simulink model "fft_biplex_real_4x_delay_bram_test"  (Simulink 7.4)
settings: Solver=VariableStepDiscrete  StartTime=0.0  StopTime=256  RelTol=1e-3
libraries: xbsIndex_r4 x596, casper_library_misc x36, casper_library_delays x8, casper_library_ffts_twiddle x1, simulink x1
(part 4 of 6)

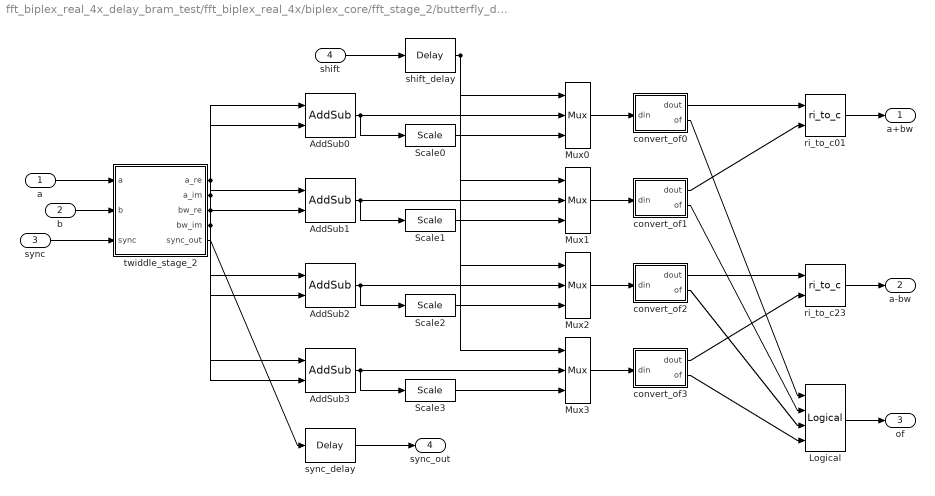
== system fft_biplex_real_4x_delay_bram_test/fft_biplex_real_4x/biplex_core/fft_stage_2/butterfly_direct ==
  a : Inport  OutDataType=sfix(16)  OutScaling=2^0
  b : Inport  Port=2  OutDataType=sfix(16)  OutScaling=2^0
  sync : Inport  Port=3  OutDataType=sfix(16)  OutScaling=2^0
  shift : Inport  Port=4  OutDataType=sfix(16)  OutScaling=2^0
  AddSub0 : xbsIndex_r4/AddSub  mode=Addition  use_carryin=off  use_carryout=off  en=off  latency=1  precision=Full  arith_type=Unsigned  n_bits=16  bin_pt=14  quantization=Truncate  overflow=Wrap  dbl_ovrd=off  use_behavioral_HDL=on  hw_selection=Fabric  pipelined=off  block_type=addsub
  AddSub1 : xbsIndex_r4/AddSub  mode=Addition  use_carryin=off  use_carryout=off  en=off  latency=1  precision=Full  arith_type=Unsigned  n_bits=16  bin_pt=14  quantization=Truncate  overflow=Wrap  dbl_ovrd=off  use_behavioral_HDL=on  hw_selection=Fabric  pipelined=off  block_type=addsub
  AddSub2 : xbsIndex_r4/AddSub  mode=Subtraction  use_carryin=off  use_carryout=off  en=off  latency=1  precision=Full  arith_type=Unsigned  n_bits=16  bin_pt=14  quantization=Truncate  overflow=Wrap  dbl_ovrd=off  use_behavioral_HDL=on  hw_selection=Fabric  pipelined=off  block_type=addsub
  AddSub3 : xbsIndex_r4/AddSub  mode=Subtraction  use_carryin=off  use_carryout=off  en=off  latency=1  precision=Full  arith_type=Unsigned  n_bits=16  bin_pt=14  quantization=Truncate  overflow=Wrap  dbl_ovrd=off  use_behavioral_HDL=on  hw_selection=Fabric  pipelined=off  block_type=addsub
  Logical : xbsIndex_r4/Logical  logical_function=OR  inputs=4  en=off  latency=0  precision=Full  arith_type=Unsigned  n_bits=16  bin_pt=0  align_bp=on  dbl_ovrd=off  block_type=logical
      settings: block_version=11.4
  Mux{0..3} (4 alike) : xbsIndex_r4/Mux  inputs=2  en=off  latency=1  precision=Full  arith_type=Unsigned  n_bits=16  bin_pt=14  quantization=Truncate  overflow=Wrap  dbl_ovrd=off  block_type=mux
      settings: block_version=11.4
  Scale{0..3} (4 alike) : xbsIndex_r4/Scale  scale_factor=-1  dbl_ovrd=off  block_type=scale
  convert_of0 : Subsystem  AncestorBlock=casper_library_misc/convert_of  mask(convert_of){bit_width_i=18, binary_point_i=16, bit_width_o=16, binary_point_o=15, latency=2, overflow=Saturate, quantization=Truncate}
      mask prompts: bit_width_i "Bit Width In"; binary_point_i "Binary Point In"; bit_width_o "Bit Width Out"; binary_point_o "Binary Point Out"; overflow "Overflow Behaviour"; quantization "Quantization Behaviour"
      mask help:
      | Converts from one 2's complement bit-width
      | and/or binary point position to another.
      | Includes underflow/overflow indicator.
      mask init: same as fft_biplex_real_4x_delay_bram_test/fft_biplex_real_4x/biplex_core/fft_stage_1/butterfly_direct/convert_of0
      settings: AttributesFormatString=[18,16]->[16,15]
      mask StyleString: edit,edit,edit,edit,edit,popup(Wrap|Saturate|Error),popup(Truncate|Round  (unbiased: +/- Inf)|Round  (unbiased: even values))
  convert_of1 : Subsystem  AncestorBlock=casper_library_misc/convert_of  mask(convert_of){bit_width_i=18, binary_point_i=16, bit_width_o=16, binary_point_o=15, latency=2, overflow=Saturate, quantization=Truncate}
      mask prompts: bit_width_i "Bit Width In"; binary_point_i "Binary Point In"; bit_width_o "Bit Width Out"; binary_point_o "Binary Point Out"; overflow "Overflow Behaviour"; quantization "Quantization Behaviour"
      mask help:
      | Converts from one 2's complement bit-width
      | and/or binary point position to another.
      | Includes underflow/overflow indicator.
      mask init: same as fft_biplex_real_4x_delay_bram_test/fft_biplex_real_4x/biplex_core/fft_stage_1/butterfly_direct/convert_of0
      settings: AttributesFormatString=[18,16]->[16,15]
      mask StyleString: edit,edit,edit,edit,edit,popup(Wrap|Saturate|Error),popup(Truncate|Round  (unbiased: +/- Inf)|Round  (unbiased: even values))
  convert_of2 : Subsystem  AncestorBlock=casper_library_misc/convert_of  mask(convert_of){bit_width_i=18, binary_point_i=16, bit_width_o=16, binary_point_o=15, latency=2, overflow=Saturate, quantization=Truncate}
      mask prompts: bit_width_i "Bit Width In"; binary_point_i "Binary Point In"; bit_width_o "Bit Width Out"; binary_point_o "Binary Point Out"; overflow "Overflow Behaviour"; quantization "Quantization Behaviour"
      mask help:
      | Converts from one 2's complement bit-width
      | and/or binary point position to another.
      | Includes underflow/overflow indicator.
      mask init: same as fft_biplex_real_4x_delay_bram_test/fft_biplex_real_4x/biplex_core/fft_stage_1/butterfly_direct/convert_of0
      settings: AttributesFormatString=[18,16]->[16,15]
      mask StyleString: edit,edit,edit,edit,edit,popup(Wrap|Saturate|Error),popup(Truncate|Round  (unbiased: +/- Inf)|Round  (unbiased: even values))
  convert_of3 : Subsystem  AncestorBlock=casper_library_misc/convert_of  mask(convert_of){bit_width_i=18, binary_point_i=16, bit_width_o=16, binary_point_o=15, latency=2, overflow=Saturate, quantization=Truncate}
      mask prompts: bit_width_i "Bit Width In"; binary_point_i "Binary Point In"; bit_width_o "Bit Width Out"; binary_point_o "Binary Point Out"; overflow "Overflow Behaviour"; quantization "Quantization Behaviour"
      mask help:
      | Converts from one 2's complement bit-width
      | and/or binary point position to another.
      | Includes underflow/overflow indicator.
      mask init: same as fft_biplex_real_4x_delay_bram_test/fft_biplex_real_4x/biplex_core/fft_stage_1/butterfly_direct/convert_of0
      settings: AttributesFormatString=[18,16]->[16,15]
      mask StyleString: edit,edit,edit,edit,edit,popup(Wrap|Saturate|Error),popup(Truncate|Round  (unbiased: +/- Inf)|Round  (unbiased: even values))
  ri_to_c01 : casper_library_misc/ri_to_c  SystemSampleTime=-1
  ri_to_c23 : casper_library_misc/ri_to_c  SystemSampleTime=-1
  shift_delay : xbsIndex_r4/Delay  en=off  latency=1  dbl_ovrd=off  reg_retiming=off  block_type=delay
      settings: block_version=11.4
  sync_delay : xbsIndex_r4/Delay  en=off  latency=4  dbl_ovrd=off  reg_retiming=on  block_type=delay
      settings: block_version=11.4
  twiddle_stage_2 : Subsystem  AncestorBlock=casper_library_ffts_twiddle/twiddle_stage_2  mask(twiddle_pass_through){FFTSize=5, input_bit_width=16, add_latency=1, mult_latency=3, bram_latency=1, conv_latency=2, opt_target=multipliers}
      mask prompts: FFTSize "FFT Size (2^?)"; input_bit_width "Input Bit Width"; add_latency "Add Latency"; mult_latency "Mult Latency"; bram_latency "BRAM Latency"; conv_latency "Convert latency"; opt_target "Use less"
      mask help:
      | Used in FFT library. Used when coefficients
      | are 2^0 i.e just pass data through without delays
      mask init:
      | set_param(gcb,'LinkStatus','inactive');
      | if(strcmp(opt_target, 'logic')), 
      |     lat = add_latency;
      |     lat_str = 'add_latency';
      | else,
      |     lat = add_latency*2;
      |     lat_str = 'add_latency*2';
      | end
      | set_param([gcb,'/delay0'], 'latency', ...
      |     ['bram_latency+mult_latency+conv_latency+',lat_str]);
      | set_param([gcb,'/delay1'], 'latency', ...
      |     ['bram_latency+mult_latency+conv_latency+',lat_str]);
      | set_param([gcb,'/mux0'], 'latency', ...
      |     num2str(mult_latency+conv_latency+lat));
      | set_param([gcb,'/mux1'], 'latency', ...
      |     num2str(mult_latency+conv_latency+lat));
      | set_param([gcb,'/delay6'], 'latency', ...
      |     ['mult_latency+conv_latency+',lat_str]);
      mask StyleString: edit,edit,edit,edit,edit,edit,popup(logic|multipliers)
  a+bw : Outport  OutDataType=sfix(16)  OutScaling=2^0
  a-bw : Outport  Port=2  OutDataType=sfix(16)  OutScaling=2^0
  of : Outport  Port=3  OutDataType=sfix(16)  OutScaling=2^0
  sync_out : Outport  Port=4
  wires:
  a/1 -> twiddle_stage_2/1(a)
  b/1 -> twiddle_stage_2/2(b)
  sync/1 -> twiddle_stage_2/3(sync)
  twiddle_stage_2/1(a_re) -> AddSub0/1, AddSub2/1
  twiddle_stage_2/2(a_im) -> AddSub1/1, AddSub3/1
  twiddle_stage_2/3(bw_re) -> AddSub0/2, AddSub2/2
  twiddle_stage_2/4(bw_im) -> AddSub1/2, AddSub3/2
  twiddle_stage_2/5(sync_out) -> sync_delay/1
  shift/1 -> shift_delay/1
  shift_delay/1 -> Mux0/1, Mux1/1, Mux2/1, Mux3/1
  AddSub0/1 -> Mux0/2, Scale0/1
  AddSub1/1 -> Mux1/2, Scale1/1
  AddSub2/1 -> Mux2/2, Scale2/1
  AddSub3/1 -> Mux3/2, Scale3/1
  Scale0/1 -> Mux0/3
  Scale1/1 -> Mux1/3
  Scale2/1 -> Mux2/3
  Scale3/1 -> Mux3/3
  Mux0/1 -> convert_of0/1(din)
  Mux1/1 -> convert_of1/1(din)
  Mux2/1 -> convert_of2/1(din)
  Mux3/1 -> convert_of3/1(din)
  convert_of0/1(dout) -> ri_to_c01/1
  convert_of1/1(dout) -> ri_to_c01/2
  convert_of2/1(dout) -> ri_to_c23/1
  convert_of3/1(dout) -> ri_to_c23/2
  convert_of0/2(of) -> Logical/1
  convert_of1/2(of) -> Logical/2
  convert_of2/2(of) -> Logical/3
  convert_of3/2(of) -> Logical/4
  ri_to_c01/1 -> a+bw/1
  ri_to_c23/1 -> a-bw/1
  Logical/1 -> of/1
  sync_delay/1 -> sync_out/1

== system fft_biplex_real_4x_delay_bram_test/fft_biplex_real_4x/biplex_core/fft_stage_2/delay_b ==
  In1 : Inport  OutDataType=sfix(16)  OutScaling=2^0
  delay_slr : xbsIndex_r4/Delay  en=off  latency=DelayLen  dbl_ovrd=off  reg_retiming=off  block_type=delay
      settings: xl_area=[0, 0, 0, 0, 0, 0, 0]  block_version=9.1.01
  Out1 : Outport  OutDataType=sfix(16)  OutScaling=2^0
  wires:
  delay_slr/1 -> Out1/1
  In1/1 -> delay_slr/1

== system fft_biplex_real_4x_delay_bram_test/fft_biplex_real_4x/biplex_core/fft_stage_2/delay_f ==
  In1 : Inport  OutDataType=sfix(16)  OutScaling=2^0
  delay_slr : xbsIndex_r4/Delay  en=off  latency=DelayLen  dbl_ovrd=off  reg_retiming=off  block_type=delay
      settings: xl_area=[0, 0, 0, 0, 0, 0, 0]  block_version=9.1.01
  Out1 : Outport  OutDataType=sfix(16)  OutScaling=2^0
  wires:
  delay_slr/1 -> Out1/1
  In1/1 -> delay_slr/1

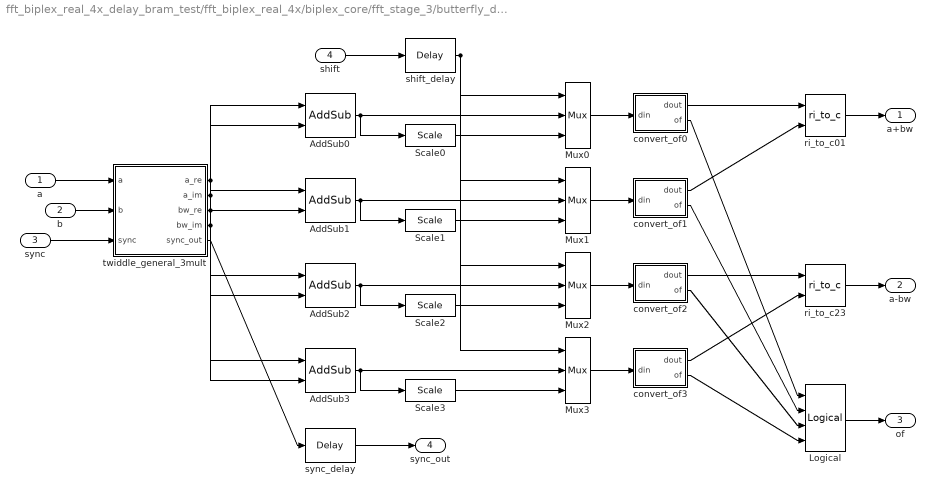
== system fft_biplex_real_4x_delay_bram_test/fft_biplex_real_4x/biplex_core/fft_stage_3/butterfly_direct ==
  a : Inport  OutDataType=sfix(16)  OutScaling=2^0
  b : Inport  Port=2  OutDataType=sfix(16)  OutScaling=2^0
  sync : Inport  Port=3  OutDataType=sfix(16)  OutScaling=2^0
  shift : Inport  Port=4  OutDataType=sfix(16)  OutScaling=2^0
  AddSub0 : xbsIndex_r4/AddSub  mode=Addition  use_carryin=off  use_carryout=off  en=off  latency=1  precision=Full  arith_type=Unsigned  n_bits=16  bin_pt=14  quantization=Truncate  overflow=Wrap  dbl_ovrd=off  use_behavioral_HDL=on  hw_selection=Fabric  pipelined=off  block_type=addsub
  AddSub1 : xbsIndex_r4/AddSub  mode=Addition  use_carryin=off  use_carryout=off  en=off  latency=1  precision=Full  arith_type=Unsigned  n_bits=16  bin_pt=14  quantization=Truncate  overflow=Wrap  dbl_ovrd=off  use_behavioral_HDL=on  hw_selection=Fabric  pipelined=off  block_type=addsub
  AddSub2 : xbsIndex_r4/AddSub  mode=Subtraction  use_carryin=off  use_carryout=off  en=off  latency=1  precision=Full  arith_type=Unsigned  n_bits=16  bin_pt=14  quantization=Truncate  overflow=Wrap  dbl_ovrd=off  use_behavioral_HDL=on  hw_selection=Fabric  pipelined=off  block_type=addsub
  AddSub3 : xbsIndex_r4/AddSub  mode=Subtraction  use_carryin=off  use_carryout=off  en=off  latency=1  precision=Full  arith_type=Unsigned  n_bits=16  bin_pt=14  quantization=Truncate  overflow=Wrap  dbl_ovrd=off  use_behavioral_HDL=on  hw_selection=Fabric  pipelined=off  block_type=addsub
  Logical : xbsIndex_r4/Logical  logical_function=OR  inputs=4  en=off  latency=0  precision=Full  arith_type=Unsigned  n_bits=16  bin_pt=0  align_bp=on  dbl_ovrd=off  block_type=logical
      settings: block_version=11.4
  Mux{0..3} (4 alike) : xbsIndex_r4/Mux  inputs=2  en=off  latency=1  precision=Full  arith_type=Unsigned  n_bits=16  bin_pt=14  quantization=Truncate  overflow=Wrap  dbl_ovrd=off  block_type=mux
      settings: block_version=11.4
  Scale{0..3} (4 alike) : xbsIndex_r4/Scale  scale_factor=-1  dbl_ovrd=off  block_type=scale
  convert_of0 : Subsystem  AncestorBlock=casper_library_misc/convert_of  mask(convert_of){bit_width_i=23, binary_point_i=18, bit_width_o=16, binary_point_o=15, latency=2, overflow=Saturate, quantization=Truncate}
      mask prompts: bit_width_i "Bit Width In"; binary_point_i "Binary Point In"; bit_width_o "Bit Width Out"; binary_point_o "Binary Point Out"; overflow "Overflow Behaviour"; quantization "Quantization Behaviour"
      mask help:
      | Converts from one 2's complement bit-width
      | and/or binary point position to another.
      | Includes underflow/overflow indicator.
      mask init: same as fft_biplex_real_4x_delay_bram_test/fft_biplex_real_4x/biplex_core/fft_stage_1/butterfly_direct/convert_of0
      settings: AttributesFormatString=[23,18]->[16,15]
      mask StyleString: edit,edit,edit,edit,edit,popup(Wrap|Saturate|Error),popup(Truncate|Round  (unbiased: +/- Inf)|Round  (unbiased: even values))
  convert_of1 : Subsystem  AncestorBlock=casper_library_misc/convert_of  mask(convert_of){bit_width_i=23, binary_point_i=18, bit_width_o=16, binary_point_o=15, latency=2, overflow=Saturate, quantization=Truncate}
      mask prompts: bit_width_i "Bit Width In"; binary_point_i "Binary Point In"; bit_width_o "Bit Width Out"; binary_point_o "Binary Point Out"; overflow "Overflow Behaviour"; quantization "Quantization Behaviour"
      mask help:
      | Converts from one 2's complement bit-width
      | and/or binary point position to another.
      | Includes underflow/overflow indicator.
      mask init: same as fft_biplex_real_4x_delay_bram_test/fft_biplex_real_4x/biplex_core/fft_stage_1/butterfly_direct/convert_of0
      settings: AttributesFormatString=[23,18]->[16,15]
      mask StyleString: edit,edit,edit,edit,edit,popup(Wrap|Saturate|Error),popup(Truncate|Round  (unbiased: +/- Inf)|Round  (unbiased: even values))
  convert_of2 : Subsystem  AncestorBlock=casper_library_misc/convert_of  mask(convert_of){bit_width_i=23, binary_point_i=18, bit_width_o=16, binary_point_o=15, latency=2, overflow=Saturate, quantization=Truncate}
      mask prompts: bit_width_i "Bit Width In"; binary_point_i "Binary Point In"; bit_width_o "Bit Width Out"; binary_point_o "Binary Point Out"; overflow "Overflow Behaviour"; quantization "Quantization Behaviour"
      mask help:
      | Converts from one 2's complement bit-width
      | and/or binary point position to another.
      | Includes underflow/overflow indicator.
      mask init: same as fft_biplex_real_4x_delay_bram_test/fft_biplex_real_4x/biplex_core/fft_stage_1/butterfly_direct/convert_of0
      settings: AttributesFormatString=[23,18]->[16,15]
      mask StyleString: edit,edit,edit,edit,edit,popup(Wrap|Saturate|Error),popup(Truncate|Round  (unbiased: +/- Inf)|Round  (unbiased: even values))
  convert_of3 : Subsystem  AncestorBlock=casper_library_misc/convert_of  mask(convert_of){bit_width_i=23, binary_point_i=18, bit_width_o=16, binary_point_o=15, latency=2, overflow=Saturate, quantization=Truncate}
      mask prompts: bit_width_i "Bit Width In"; binary_point_i "Binary Point In"; bit_width_o "Bit Width Out"; binary_point_o "Binary Point Out"; overflow "Overflow Behaviour"; quantization "Quantization Behaviour"
      mask help:
      | Converts from one 2's complement bit-width
      | and/or binary point position to another.
      | Includes underflow/overflow indicator.
      mask init: same as fft_biplex_real_4x_delay_bram_test/fft_biplex_real_4x/biplex_core/fft_stage_1/butterfly_direct/convert_of0
      settings: AttributesFormatString=[23,18]->[16,15]
      mask StyleString: edit,edit,edit,edit,edit,popup(Wrap|Saturate|Error),popup(Truncate|Round  (unbiased: +/- Inf)|Round  (unbiased: even values))
  ri_to_c01 : casper_library_misc/ri_to_c  SystemSampleTime=-1
  ri_to_c23 : casper_library_misc/ri_to_c  SystemSampleTime=-1
  shift_delay : xbsIndex_r4/Delay  en=off  latency=1  dbl_ovrd=off  reg_retiming=off  block_type=delay
      settings: block_version=11.4
  sync_delay : xbsIndex_r4/Delay  en=off  latency=4  dbl_ovrd=off  reg_retiming=on  block_type=delay
      settings: block_version=11.4
  twiddle_general_3mult : Subsystem  AncestorBlock=casper_library_ffts_twiddle/twiddle_general_3mult  mask(twiddle_general_3mult){Coeffs=getfield( getfield( get_param( gcb,'UserData' ), 'parameters'),'Coeffs'), StepPeriod=2, coeffs_bram=off, coeff_bit_width=16, input_bit_width=16, add_latency=1, mult_latency=3, bram_latency=1, conv_latency=2, arch=Virtex2Pro, use_hdl=on, use_embedded=off, quantization=Truncate, overflow=Saturate}
      mask prompts: Coeffs "Coefficients:"; StepPeriod "Coefficient Step Period (2^?)"; coeffs_bram "Store coefficients in BRAM"; coeff_bit_width "Coefficient Bit Width"; input_bit_width "Input Bit Width"; add_latency "Add Latency"; mult_latency "Mult Latency"; bram_latency "BRAM Latency"; conv_latency "Convert latency"; arch "Architecture"; use_hdl "Use behavioral HDL for multlipliers"; use_embedded "Use embedded multipliers"; quantization "Quantization Behavior"; overflow "Overflow Behavior"
      mask help:
      | Used in biplex pipelined FFT. Takes advantage that
      | (a+bi)(c+di)=(c(a+b)-b(c+d))+i(b(c+d)+a(c-d)) to
      | save on multipliers at expense of adders.
      mask init:
      | twiddle_general_3mult_init(gcb, ... 
      |     'Coeffs', Coeffs, ...
      |     'StepPeriod', StepPeriod, ...
      |     'coeffs_bram', coeffs_bram, ...
      |     'coeff_bit_width', coeff_bit_width, ...
      |     'input_bit_width', input_bit_width, ...
      |     'add_latency', add_latency, ...
      |     'mult_latency', mult_latency, ...
      |     'bram_latency', bram_latency, ...
      |     'conv_latency', conv_latency, ...
      |     'arch', arch, 'use_hdl', use_hdl, ...
      |     'use_embedded', use_embedded, ...
      |     'quantization', quantization, ...
      |     'overflow', overflow)
      settings: AttributesFormatString=|
      | data=(16,15)
      | coeffs=(15,13)
      | Virtex2Pro
      | (Truncate,Saturate)
      mask StyleString: edit,edit,checkbox,edit,edit,edit,edit,edit,edit,popup(Virtex2Pro|Virtex5),checkbox,checkbox,popup(Truncate|Round  (unbiased: +/- Inf)|Round  (unbiased: Even Values)),popup(Wrap|Saturate|Error)
      mask CallbackString:
      | ||||||||||use_hdl = get_param(gcb,'use_hdl');
      | visibs = get_param(gcb, 'MaskVisibilities');
      | if( strcmp(use_hdl,'on')),
      |     set_param(gcb, 'use_embedded','off');
      |     visibs{12} = 'off';
      | else,
      |     visibs{12} = 'on';
      | end
      | set_param(gcb, 'MaskVisibilities', visibs);
      | |||
  a+bw : Outport  OutDataType=sfix(16)  OutScaling=2^0
  a-bw : Outport  Port=2  OutDataType=sfix(16)  OutScaling=2^0
  of : Outport  Port=3  OutDataType=sfix(16)  OutScaling=2^0
  sync_out : Outport  Port=4
  wires:
  a/1 -> twiddle_general_3mult/1(a)
  b/1 -> twiddle_general_3mult/2(b)
  sync/1 -> twiddle_general_3mult/3(sync)
  twiddle_general_3mult/1(a_re) -> AddSub0/1, AddSub2/1
  twiddle_general_3mult/2(a_im) -> AddSub1/1, AddSub3/1
  twiddle_general_3mult/3(bw_re) -> AddSub0/2, AddSub2/2
  twiddle_general_3mult/4(bw_im) -> AddSub1/2, AddSub3/2
  twiddle_general_3mult/5(sync_out) -> sync_delay/1
  shift/1 -> shift_delay/1
  shift_delay/1 -> Mux0/1, Mux1/1, Mux2/1, Mux3/1
  AddSub0/1 -> Mux0/2, Scale0/1
  AddSub1/1 -> Mux1/2, Scale1/1
  AddSub2/1 -> Mux2/2, Scale2/1
  AddSub3/1 -> Mux3/2, Scale3/1
  Scale0/1 -> Mux0/3
  Scale1/1 -> Mux1/3
  Scale2/1 -> Mux2/3
  Scale3/1 -> Mux3/3
  Mux0/1 -> convert_of0/1(din)
  Mux1/1 -> convert_of1/1(din)
  Mux2/1 -> convert_of2/1(din)
  Mux3/1 -> convert_of3/1(din)
  convert_of0/1(dout) -> ri_to_c01/1
  convert_of1/1(dout) -> ri_to_c01/2
  convert_of2/1(dout) -> ri_to_c23/1
  convert_of3/1(dout) -> ri_to_c23/2
  convert_of0/2(of) -> Logical/1
  convert_of1/2(of) -> Logical/2
  convert_of2/2(of) -> Logical/3
  convert_of3/2(of) -> Logical/4
  ri_to_c01/1 -> a+bw/1
  ri_to_c23/1 -> a-bw/1
  Logical/1 -> of/1
  sync_delay/1 -> sync_out/1

== system fft_biplex_real_4x_delay_bram_test/fft_biplex_real_4x/biplex_core/fft_stage_3/delay_b ==
  In1 : Inport  OutDataType=sfix(16)  OutScaling=2^0
  delay_slr : xbsIndex_r4/Delay  en=off  latency=DelayLen  dbl_ovrd=off  reg_retiming=off  block_type=delay
      settings: xl_area=[0, 0, 0, 0, 0, 0, 0]  block_version=9.1.01
  Out1 : Outport  OutDataType=sfix(16)  OutScaling=2^0
  wires:
  delay_slr/1 -> Out1/1
  In1/1 -> delay_slr/1

== system fft_biplex_real_4x_delay_bram_test/fft_biplex_real_4x/biplex_core/fft_stage_3/delay_f ==
  In1 : Inport  OutDataType=sfix(16)  OutScaling=2^0
  delay_slr : xbsIndex_r4/Delay  en=off  latency=DelayLen  dbl_ovrd=off  reg_retiming=off  block_type=delay
      settings: xl_area=[0, 0, 0, 0, 0, 0, 0]  block_version=9.1.01
  Out1 : Outport  OutDataType=sfix(16)  OutScaling=2^0
  wires:
  delay_slr/1 -> Out1/1
  In1/1 -> delay_slr/1

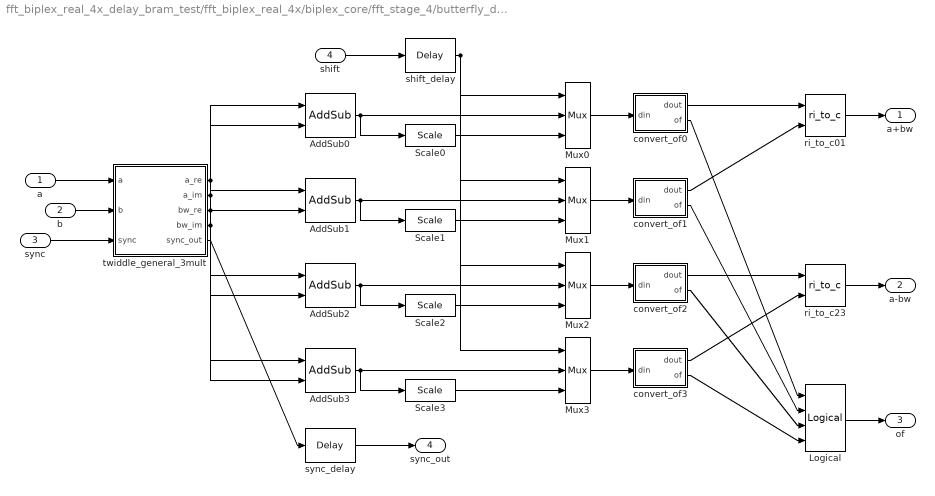
== system fft_biplex_real_4x_delay_bram_test/fft_biplex_real_4x/biplex_core/fft_stage_4/butterfly_direct ==
  a : Inport  OutDataType=sfix(16)  OutScaling=2^0
  b : Inport  Port=2  OutDataType=sfix(16)  OutScaling=2^0
  sync : Inport  Port=3  OutDataType=sfix(16)  OutScaling=2^0
  shift : Inport  Port=4  OutDataType=sfix(16)  OutScaling=2^0
  AddSub0 : xbsIndex_r4/AddSub  mode=Addition  use_carryin=off  use_carryout=off  en=off  latency=1  precision=Full  arith_type=Unsigned  n_bits=16  bin_pt=14  quantization=Truncate  overflow=Wrap  dbl_ovrd=off  use_behavioral_HDL=on  hw_selection=Fabric  pipelined=off  block_type=addsub
  AddSub1 : xbsIndex_r4/AddSub  mode=Addition  use_carryin=off  use_carryout=off  en=off  latency=1  precision=Full  arith_type=Unsigned  n_bits=16  bin_pt=14  quantization=Truncate  overflow=Wrap  dbl_ovrd=off  use_behavioral_HDL=on  hw_selection=Fabric  pipelined=off  block_type=addsub
  AddSub2 : xbsIndex_r4/AddSub  mode=Subtraction  use_carryin=off  use_carryout=off  en=off  latency=1  precision=Full  arith_type=Unsigned  n_bits=16  bin_pt=14  quantization=Truncate  overflow=Wrap  dbl_ovrd=off  use_behavioral_HDL=on  hw_selection=Fabric  pipelined=off  block_type=addsub
  AddSub3 : xbsIndex_r4/AddSub  mode=Subtraction  use_carryin=off  use_carryout=off  en=off  latency=1  precision=Full  arith_type=Unsigned  n_bits=16  bin_pt=14  quantization=Truncate  overflow=Wrap  dbl_ovrd=off  use_behavioral_HDL=on  hw_selection=Fabric  pipelined=off  block_type=addsub
  Logical : xbsIndex_r4/Logical  logical_function=OR  inputs=4  en=off  latency=0  precision=Full  arith_type=Unsigned  n_bits=16  bin_pt=0  align_bp=on  dbl_ovrd=off  block_type=logical
      settings: block_version=11.4
  Mux{0..3} (4 alike) : xbsIndex_r4/Mux  inputs=2  en=off  latency=1  precision=Full  arith_type=Unsigned  n_bits=16  bin_pt=14  quantization=Truncate  overflow=Wrap  dbl_ovrd=off  block_type=mux
      settings: block_version=11.4
  Scale{0..3} (4 alike) : xbsIndex_r4/Scale  scale_factor=-1  dbl_ovrd=off  block_type=scale
  convert_of0 : Subsystem  AncestorBlock=casper_library_misc/convert_of  mask(convert_of){bit_width_i=23, binary_point_i=18, bit_width_o=16, binary_point_o=15, latency=2, overflow=Saturate, quantization=Truncate}
      mask prompts: bit_width_i "Bit Width In"; binary_point_i "Binary Point In"; bit_width_o "Bit Width Out"; binary_point_o "Binary Point Out"; overflow "Overflow Behaviour"; quantization "Quantization Behaviour"
      mask help:
      | Converts from one 2's complement bit-width
      | and/or binary point position to another.
      | Includes underflow/overflow indicator.
      mask init: same as fft_biplex_real_4x_delay_bram_test/fft_biplex_real_4x/biplex_core/fft_stage_1/butterfly_direct/convert_of0
      settings: AttributesFormatString=[23,18]->[16,15]
      mask StyleString: edit,edit,edit,edit,edit,popup(Wrap|Saturate|Error),popup(Truncate|Round  (unbiased: +/- Inf)|Round  (unbiased: even values))
  convert_of1 : Subsystem  AncestorBlock=casper_library_misc/convert_of  mask(convert_of){bit_width_i=23, binary_point_i=18, bit_width_o=16, binary_point_o=15, latency=2, overflow=Saturate, quantization=Truncate}
      mask prompts: bit_width_i "Bit Width In"; binary_point_i "Binary Point In"; bit_width_o "Bit Width Out"; binary_point_o "Binary Point Out"; overflow "Overflow Behaviour"; quantization "Quantization Behaviour"
      mask help:
      | Converts from one 2's complement bit-width
      | and/or binary point position to another.
      | Includes underflow/overflow indicator.
      mask init: same as fft_biplex_real_4x_delay_bram_test/fft_biplex_real_4x/biplex_core/fft_stage_1/butterfly_direct/convert_of0
      settings: AttributesFormatString=[23,18]->[16,15]
      mask StyleString: edit,edit,edit,edit,edit,popup(Wrap|Saturate|Error),popup(Truncate|Round  (unbiased: +/- Inf)|Round  (unbiased: even values))
  convert_of2 : Subsystem  AncestorBlock=casper_library_misc/convert_of  mask(convert_of){bit_width_i=23, binary_point_i=18, bit_width_o=16, binary_point_o=15, latency=2, overflow=Saturate, quantization=Truncate}
      mask prompts: bit_width_i "Bit Width In"; binary_point_i "Binary Point In"; bit_width_o "Bit Width Out"; binary_point_o "Binary Point Out"; overflow "Overflow Behaviour"; quantization "Quantization Behaviour"
      mask help:
      | Converts from one 2's complement bit-width
      | and/or binary point position to another.
      | Includes underflow/overflow indicator.
      mask init: same as fft_biplex_real_4x_delay_bram_test/fft_biplex_real_4x/biplex_core/fft_stage_1/butterfly_direct/convert_of0
      settings: AttributesFormatString=[23,18]->[16,15]
      mask StyleString: edit,edit,edit,edit,edit,popup(Wrap|Saturate|Error),popup(Truncate|Round  (unbiased: +/- Inf)|Round  (unbiased: even values))
  convert_of3 : Subsystem  AncestorBlock=casper_library_misc/convert_of  mask(convert_of){bit_width_i=23, binary_point_i=18, bit_width_o=16, binary_point_o=15, latency=2, overflow=Saturate, quantization=Truncate}
      mask prompts: bit_width_i "Bit Width In"; binary_point_i "Binary Point In"; bit_width_o "Bit Width Out"; binary_point_o "Binary Point Out"; overflow "Overflow Behaviour"; quantization "Quantization Behaviour"
      mask help:
      | Converts from one 2's complement bit-width
      | and/or binary point position to another.
      | Includes underflow/overflow indicator.
      mask init: same as fft_biplex_real_4x_delay_bram_test/fft_biplex_real_4x/biplex_core/fft_stage_1/butterfly_direct/convert_of0
      settings: AttributesFormatString=[23,18]->[16,15]
      mask StyleString: edit,edit,edit,edit,edit,popup(Wrap|Saturate|Error),popup(Truncate|Round  (unbiased: +/- Inf)|Round  (unbiased: even values))
  ri_to_c01 : casper_library_misc/ri_to_c  SystemSampleTime=-1
  ri_to_c23 : casper_library_misc/ri_to_c  SystemSampleTime=-1
  shift_delay : xbsIndex_r4/Delay  en=off  latency=1  dbl_ovrd=off  reg_retiming=off  block_type=delay
      settings: block_version=11.4
  sync_delay : xbsIndex_r4/Delay  en=off  latency=4  dbl_ovrd=off  reg_retiming=on  block_type=delay
      settings: block_version=11.4
  twiddle_general_3mult : Subsystem  AncestorBlock=casper_library_ffts_twiddle/twiddle_general_3mult  mask(twiddle_general_3mult){Coeffs=getfield( getfield( get_param( gcb,'UserData' ), 'parameters'),'Coeffs'), StepPeriod=1, coeffs_bram=off, coeff_bit_width=16, input_bit_width=16, add_latency=1, mult_latency=3, bram_latency=1, conv_latency=2, arch=Virtex2Pro, use_hdl=on, use_embedded=off, quantization=Truncate, overflow=Saturate}
      mask prompts: Coeffs "Coefficients:"; StepPeriod "Coefficient Step Period (2^?)"; coeffs_bram "Store coefficients in BRAM"; coeff_bit_width "Coefficient Bit Width"; input_bit_width "Input Bit Width"; add_latency "Add Latency"; mult_latency "Mult Latency"; bram_latency "BRAM Latency"; conv_latency "Convert latency"; arch "Architecture"; use_hdl "Use behavioral HDL for multlipliers"; use_embedded "Use embedded multipliers"; quantization "Quantization Behavior"; overflow "Overflow Behavior"
      mask help:
      | Used in biplex pipelined FFT. Takes advantage that
      | (a+bi)(c+di)=(c(a+b)-b(c+d))+i(b(c+d)+a(c-d)) to
      | save on multipliers at expense of adders.
      mask init: same as fft_biplex_real_4x_delay_bram_test/fft_biplex_real_4x/biplex_core/fft_stage_3/butterfly_direct/twiddle_general_3mult
      settings: AttributesFormatString=|
      | data=(16,15)
      | coeffs=(15,13)
      | Virtex2Pro
      | (Truncate,Saturate)
      mask StyleString: edit,edit,checkbox,edit,edit,edit,edit,edit,edit,popup(Virtex2Pro|Virtex5),checkbox,checkbox,popup(Truncate|Round  (unbiased: +/- Inf)|Round  (unbiased: Even Values)),popup(Wrap|Saturate|Error)
      mask CallbackString:
      | ||||||||||use_hdl = get_param(gcb,'use_hdl');
      | visibs = get_param(gcb, 'MaskVisibilities');
      | if( strcmp(use_hdl,'on')),
      |     set_param(gcb, 'use_embedded','off');
      |     visibs{12} = 'off';
      | else,
      |     visibs{12} = 'on';
      | end
      | set_param(gcb, 'MaskVisibilities', visibs);
      | |||
  a+bw : Outport  OutDataType=sfix(16)  OutScaling=2^0
  a-bw : Outport  Port=2  OutDataType=sfix(16)  OutScaling=2^0
  of : Outport  Port=3  OutDataType=sfix(16)  OutScaling=2^0
  sync_out : Outport  Port=4
  wires:
  a/1 -> twiddle_general_3mult/1(a)
  b/1 -> twiddle_general_3mult/2(b)
  sync/1 -> twiddle_general_3mult/3(sync)
  twiddle_general_3mult/1(a_re) -> AddSub0/1, AddSub2/1
  twiddle_general_3mult/2(a_im) -> AddSub1/1, AddSub3/1
  twiddle_general_3mult/3(bw_re) -> AddSub0/2, AddSub2/2
  twiddle_general_3mult/4(bw_im) -> AddSub1/2, AddSub3/2
  twiddle_general_3mult/5(sync_out) -> sync_delay/1
  shift/1 -> shift_delay/1
  shift_delay/1 -> Mux0/1, Mux1/1, Mux2/1, Mux3/1
  AddSub0/1 -> Mux0/2, Scale0/1
  AddSub1/1 -> Mux1/2, Scale1/1
  AddSub2/1 -> Mux2/2, Scale2/1
  AddSub3/1 -> Mux3/2, Scale3/1
  Scale0/1 -> Mux0/3
  Scale1/1 -> Mux1/3
  Scale2/1 -> Mux2/3
  Scale3/1 -> Mux3/3
  Mux0/1 -> convert_of0/1(din)
  Mux1/1 -> convert_of1/1(din)
  Mux2/1 -> convert_of2/1(din)
  Mux3/1 -> convert_of3/1(din)
  convert_of0/1(dout) -> ri_to_c01/1
  convert_of1/1(dout) -> ri_to_c01/2
  convert_of2/1(dout) -> ri_to_c23/1
  convert_of3/1(dout) -> ri_to_c23/2
  convert_of0/2(of) -> Logical/1
  convert_of1/2(of) -> Logical/2
  convert_of2/2(of) -> Logical/3
  convert_of3/2(of) -> Logical/4
  ri_to_c01/1 -> a+bw/1
  ri_to_c23/1 -> a-bw/1
  Logical/1 -> of/1
  sync_delay/1 -> sync_out/1

== system fft_biplex_real_4x_delay_bram_test/fft_biplex_real_4x/biplex_core/fft_stage_4/delay_b ==
  In1 : Inport  OutDataType=sfix(16)  OutScaling=2^0
  delay_slr : xbsIndex_r4/Delay  en=off  latency=DelayLen  dbl_ovrd=off  reg_retiming=off  block_type=delay
      settings: xl_area=[0, 0, 0, 0, 0, 0, 0]  block_version=9.1.01
  Out1 : Outport  OutDataType=sfix(16)  OutScaling=2^0
  wires:
  delay_slr/1 -> Out1/1
  In1/1 -> delay_slr/1

== system fft_biplex_real_4x_delay_bram_test/fft_biplex_real_4x/biplex_core/fft_stage_4/delay_f ==
  In1 : Inport  OutDataType=sfix(16)  OutScaling=2^0
  delay_slr : xbsIndex_r4/Delay  en=off  latency=DelayLen  dbl_ovrd=off  reg_retiming=off  block_type=delay
      settings: xl_area=[0, 0, 0, 0, 0, 0, 0]  block_version=9.1.01
  Out1 : Outport  OutDataType=sfix(16)  OutScaling=2^0
  wires:
  delay_slr/1 -> Out1/1
  In1/1 -> delay_slr/1

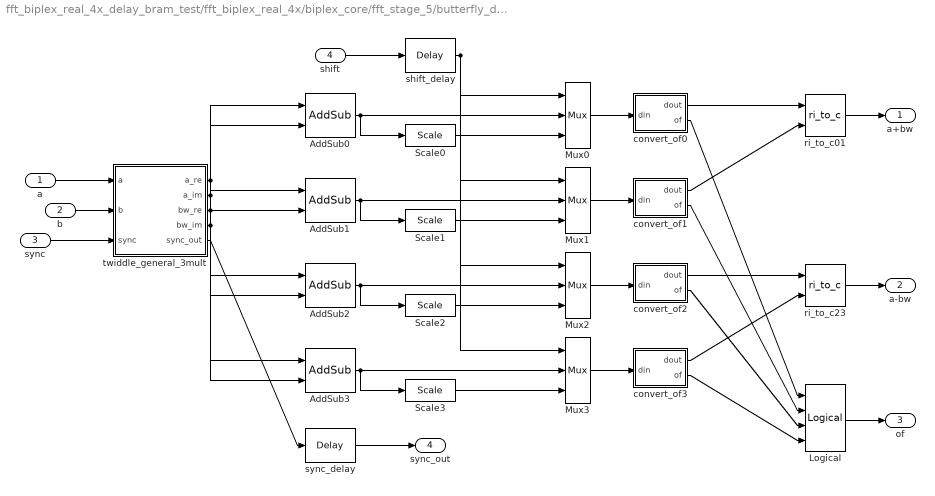
== system fft_biplex_real_4x_delay_bram_test/fft_biplex_real_4x/biplex_core/fft_stage_5/butterfly_direct ==
  a : Inport  OutDataType=sfix(16)  OutScaling=2^0
  b : Inport  Port=2  OutDataType=sfix(16)  OutScaling=2^0
  sync : Inport  Port=3  OutDataType=sfix(16)  OutScaling=2^0
  shift : Inport  Port=4  OutDataType=sfix(16)  OutScaling=2^0
  AddSub0 : xbsIndex_r4/AddSub  mode=Addition  use_carryin=off  use_carryout=off  en=off  latency=1  precision=Full  arith_type=Unsigned  n_bits=16  bin_pt=14  quantization=Truncate  overflow=Wrap  dbl_ovrd=off  use_behavioral_HDL=on  hw_selection=Fabric  pipelined=off  block_type=addsub
  AddSub1 : xbsIndex_r4/AddSub  mode=Addition  use_carryin=off  use_carryout=off  en=off  latency=1  precision=Full  arith_type=Unsigned  n_bits=16  bin_pt=14  quantization=Truncate  overflow=Wrap  dbl_ovrd=off  use_behavioral_HDL=on  hw_selection=Fabric  pipelined=off  block_type=addsub
  AddSub2 : xbsIndex_r4/AddSub  mode=Subtraction  use_carryin=off  use_carryout=off  en=off  latency=1  precision=Full  arith_type=Unsigned  n_bits=16  bin_pt=14  quantization=Truncate  overflow=Wrap  dbl_ovrd=off  use_behavioral_HDL=on  hw_selection=Fabric  pipelined=off  block_type=addsub
  AddSub3 : xbsIndex_r4/AddSub  mode=Subtraction  use_carryin=off  use_carryout=off  en=off  latency=1  precision=Full  arith_type=Unsigned  n_bits=16  bin_pt=14  quantization=Truncate  overflow=Wrap  dbl_ovrd=off  use_behavioral_HDL=on  hw_selection=Fabric  pipelined=off  block_type=addsub
  Logical : xbsIndex_r4/Logical  logical_function=OR  inputs=4  en=off  latency=0  precision=Full  arith_type=Unsigned  n_bits=16  bin_pt=0  align_bp=on  dbl_ovrd=off  block_type=logical
      settings: block_version=11.4
  Mux{0..3} (4 alike) : xbsIndex_r4/Mux  inputs=2  en=off  latency=1  precision=Full  arith_type=Unsigned  n_bits=16  bin_pt=14  quantization=Truncate  overflow=Wrap  dbl_ovrd=off  block_type=mux
      settings: block_version=11.4
  Scale{0..3} (4 alike) : xbsIndex_r4/Scale  scale_factor=-1  dbl_ovrd=off  block_type=scale
  convert_of0 : Subsystem  AncestorBlock=casper_library_misc/convert_of  mask(convert_of){bit_width_i=23, binary_point_i=18, bit_width_o=16, binary_point_o=15, latency=2, overflow=Saturate, quantization=Truncate}
      mask prompts: bit_width_i "Bit Width In"; binary_point_i "Binary Point In"; bit_width_o "Bit Width Out"; binary_point_o "Binary Point Out"; overflow "Overflow Behaviour"; quantization "Quantization Behaviour"
      mask help:
      | Converts from one 2's complement bit-width
      | and/or binary point position to another.
      | Includes underflow/overflow indicator.
      mask init: same as fft_biplex_real_4x_delay_bram_test/fft_biplex_real_4x/biplex_core/fft_stage_1/butterfly_direct/convert_of0
      settings: AttributesFormatString=[23,18]->[16,15]
      mask StyleString: edit,edit,edit,edit,edit,popup(Wrap|Saturate|Error),popup(Truncate|Round  (unbiased: +/- Inf)|Round  (unbiased: even values))
  convert_of1 : Subsystem  AncestorBlock=casper_library_misc/convert_of  mask(convert_of){bit_width_i=23, binary_point_i=18, bit_width_o=16, binary_point_o=15, latency=2, overflow=Saturate, quantization=Truncate}
      mask prompts: bit_width_i "Bit Width In"; binary_point_i "Binary Point In"; bit_width_o "Bit Width Out"; binary_point_o "Binary Point Out"; overflow "Overflow Behaviour"; quantization "Quantization Behaviour"
      mask help:
      | Converts from one 2's complement bit-width
      | and/or binary point position to another.
      | Includes underflow/overflow indicator.
      mask init: same as fft_biplex_real_4x_delay_bram_test/fft_biplex_real_4x/biplex_core/fft_stage_1/butterfly_direct/convert_of0
      settings: AttributesFormatString=[23,18]->[16,15]
      mask StyleString: edit,edit,edit,edit,edit,popup(Wrap|Saturate|Error),popup(Truncate|Round  (unbiased: +/- Inf)|Round  (unbiased: even values))
  convert_of2 : Subsystem  AncestorBlock=casper_library_misc/convert_of  mask(convert_of){bit_width_i=23, binary_point_i=18, bit_width_o=16, binary_point_o=15, latency=2, overflow=Saturate, quantization=Truncate}
      mask prompts: bit_width_i "Bit Width In"; binary_point_i "Binary Point In"; bit_width_o "Bit Width Out"; binary_point_o "Binary Point Out"; overflow "Overflow Behaviour"; quantization "Quantization Behaviour"
      mask help:
      | Converts from one 2's complement bit-width
      | and/or binary point position to another.
      | Includes underflow/overflow indicator.
      mask init: same as fft_biplex_real_4x_delay_bram_test/fft_biplex_real_4x/biplex_core/fft_stage_1/butterfly_direct/convert_of0
      settings: AttributesFormatString=[23,18]->[16,15]
      mask StyleString: edit,edit,edit,edit,edit,popup(Wrap|Saturate|Error),popup(Truncate|Round  (unbiased: +/- Inf)|Round  (unbiased: even values))
  convert_of3 : Subsystem  AncestorBlock=casper_library_misc/convert_of  mask(convert_of){bit_width_i=23, binary_point_i=18, bit_width_o=16, binary_point_o=15, latency=2, overflow=Saturate, quantization=Truncate}
      mask prompts: bit_width_i "Bit Width In"; binary_point_i "Binary Point In"; bit_width_o "Bit Width Out"; binary_point_o "Binary Point Out"; overflow "Overflow Behaviour"; quantization "Quantization Behaviour"
      mask help:
      | Converts from one 2's complement bit-width
      | and/or binary point position to another.
      | Includes underflow/overflow indicator.
      mask init: same as fft_biplex_real_4x_delay_bram_test/fft_biplex_real_4x/biplex_core/fft_stage_1/butterfly_direct/convert_of0
      settings: AttributesFormatString=[23,18]->[16,15]
      mask StyleString: edit,edit,edit,edit,edit,popup(Wrap|Saturate|Error),popup(Truncate|Round  (unbiased: +/- Inf)|Round  (unbiased: even values))
  ri_to_c01 : casper_library_misc/ri_to_c  SystemSampleTime=-1
  ri_to_c23 : casper_library_misc/ri_to_c  SystemSampleTime=-1
  shift_delay : xbsIndex_r4/Delay  en=off  latency=1  dbl_ovrd=off  reg_retiming=off  block_type=delay
      settings: block_version=11.4
  sync_delay : xbsIndex_r4/Delay  en=off  latency=4  dbl_ovrd=off  reg_retiming=on  block_type=delay
      settings: block_version=11.4
  twiddle_general_3mult : Subsystem  AncestorBlock=casper_library_ffts_twiddle/twiddle_general_3mult  mask(twiddle_general_3mult){Coeffs=getfield( getfield( get_param( gcb,'UserData' ), 'parameters'),'Coeffs'), StepPeriod=0, coeffs_bram=off, coeff_bit_width=16, input_bit_width=16, add_latency=1, mult_latency=3, bram_latency=1, conv_latency=2, arch=Virtex2Pro, use_hdl=off, use_embedded=on, quantization=Truncate, overflow=Saturate}
      mask prompts: Coeffs "Coefficients:"; StepPeriod "Coefficient Step Period (2^?)"; coeffs_bram "Store coefficients in BRAM"; coeff_bit_width "Coefficient Bit Width"; input_bit_width "Input Bit Width"; add_latency "Add Latency"; mult_latency "Mult Latency"; bram_latency "BRAM Latency"; conv_latency "Convert latency"; arch "Architecture"; use_hdl "Use behavioral HDL for multlipliers"; use_embedded "Use embedded multipliers"; quantization "Quantization Behavior"; overflow "Overflow Behavior"
      mask help:
      | Used in biplex pipelined FFT. Takes advantage that
      | (a+bi)(c+di)=(c(a+b)-b(c+d))+i(b(c+d)+a(c-d)) to
      | save on multipliers at expense of adders.
      mask init: same as fft_biplex_real_4x_delay_bram_test/fft_biplex_real_4x/biplex_core/fft_stage_3/butterfly_direct/twiddle_general_3mult
      settings: AttributesFormatString=|
      | data=(16,15)
      | coeffs=(15,13)
      | Virtex2Pro
      | (Truncate,Saturate)
      mask StyleString: edit,edit,checkbox,edit,edit,edit,edit,edit,edit,popup(Virtex2Pro|Virtex5),checkbox,checkbox,popup(Truncate|Round  (unbiased: +/- Inf)|Round  (unbiased: Even Values)),popup(Wrap|Saturate|Error)
      mask CallbackString:
      | ||||||||||use_hdl = get_param(gcb,'use_hdl');
      | visibs = get_param(gcb, 'MaskVisibilities');
      | if( strcmp(use_hdl,'on')),
      |     set_param(gcb, 'use_embedded','off');
      |     visibs{12} = 'off';
      | else,
      |     visibs{12} = 'on';
      | end
      | set_param(gcb, 'MaskVisibilities', visibs);
      | |||
  a+bw : Outport  OutDataType=sfix(16)  OutScaling=2^0
  a-bw : Outport  Port=2  OutDataType=sfix(16)  OutScaling=2^0
  of : Outport  Port=3  OutDataType=sfix(16)  OutScaling=2^0
  sync_out : Outport  Port=4
  wires:
  a/1 -> twiddle_general_3mult/1(a)
  b/1 -> twiddle_general_3mult/2(b)
  sync/1 -> twiddle_general_3mult/3(sync)
  twiddle_general_3mult/1(a_re) -> AddSub0/1, AddSub2/1
  twiddle_general_3mult/2(a_im) -> AddSub1/1, AddSub3/1
  twiddle_general_3mult/3(bw_re) -> AddSub0/2, AddSub2/2
  twiddle_general_3mult/4(bw_im) -> AddSub1/2, AddSub3/2
  twiddle_general_3mult/5(sync_out) -> sync_delay/1
  shift/1 -> shift_delay/1
  shift_delay/1 -> Mux0/1, Mux1/1, Mux2/1, Mux3/1
  AddSub0/1 -> Mux0/2, Scale0/1
  AddSub1/1 -> Mux1/2, Scale1/1
  AddSub2/1 -> Mux2/2, Scale2/1
  AddSub3/1 -> Mux3/2, Scale3/1
  Scale0/1 -> Mux0/3
  Scale1/1 -> Mux1/3
  Scale2/1 -> Mux2/3
  Scale3/1 -> Mux3/3
  Mux0/1 -> convert_of0/1(din)
  Mux1/1 -> convert_of1/1(din)
  Mux2/1 -> convert_of2/1(din)
  Mux3/1 -> convert_of3/1(din)
  convert_of0/1(dout) -> ri_to_c01/1
  convert_of1/1(dout) -> ri_to_c01/2
  convert_of2/1(dout) -> ri_to_c23/1
  convert_of3/1(dout) -> ri_to_c23/2
  convert_of0/2(of) -> Logical/1
  convert_of1/2(of) -> Logical/2
  convert_of2/2(of) -> Logical/3
  convert_of3/2(of) -> Logical/4
  ri_to_c01/1 -> a+bw/1
  ri_to_c23/1 -> a-bw/1
  Logical/1 -> of/1
  sync_delay/1 -> sync_out/1

== system fft_biplex_real_4x_delay_bram_test/fft_biplex_real_4x/biplex_core/fft_stage_5/delay_b ==
  In1 : Inport  OutDataType=sfix(16)  OutScaling=2^0
  delay_slr : xbsIndex_r4/Delay  en=off  latency=DelayLen  dbl_ovrd=off  reg_retiming=off  block_type=delay
      settings: xl_area=[0, 0, 0, 0, 0, 0, 0]  block_version=9.1.01
  Out1 : Outport  OutDataType=sfix(16)  OutScaling=2^0
  wires:
  delay_slr/1 -> Out1/1
  In1/1 -> delay_slr/1

== system fft_biplex_real_4x_delay_bram_test/fft_biplex_real_4x/biplex_core/fft_stage_5/delay_f ==
  In1 : Inport  OutDataType=sfix(16)  OutScaling=2^0
  delay_slr : xbsIndex_r4/Delay  en=off  latency=DelayLen  dbl_ovrd=off  reg_retiming=off  block_type=delay
      settings: xl_area=[0, 0, 0, 0, 0, 0, 0]  block_version=9.1.01
  Out1 : Outport  OutDataType=sfix(16)  OutScaling=2^0
  wires:
  delay_slr/1 -> Out1/1
  In1/1 -> delay_slr/1

== system fft_biplex_real_4x_delay_bram_test/fft_biplex_real_4x/biplex_core/fft_stage_1/butterfly_direct/convert_of0 ==
  din : Inport  OutDataType=sfix(16)  OutScaling=2^0
  all_0s : xbsIndex_r4/Logical  logical_function=NAND  inputs=2  en=off  latency=latency  precision=Full  arith_type=Unsigned  n_bits=16  bin_pt=0  align_bp=on  dbl_ovrd=off  block_type=logical
  all_1s : xbsIndex_r4/Logical  logical_function=NAND  inputs=2  en=off  latency=latency  precision=Full  arith_type=Unsigned  n_bits=16  bin_pt=0  align_bp=on  dbl_ovrd=off  block_type=logical
  and : xbsIndex_r4/Logical  logical_function=AND  inputs=2  en=off  latency=0  precision=Full  arith_type=Unsigned  n_bits=16  bin_pt=0  align_bp=on  dbl_ovrd=off  block_type=logical
  convert : xbsIndex_r4/Convert  arith_type="Signed  (2's comp)"  n_bits=bit_width_o  bin_pt=binary_point_o  quantization=Truncate  overflow=Saturate  latency=latency  dbl_ovrd=off  pipeline=on  block_type=convert
      settings: block_version=10.1.1
  invert1 : xbsIndex_r4/Inverter  en=off  latency=0  dbl_ovrd=off  block_type=inv
  invert2 : xbsIndex_r4/Inverter  en=off  latency=0  dbl_ovrd=off  block_type=inv
  slice1 : xbsIndex_r4/Slice  nbits=1  boolean_output=on  mode=Upper Bit Location + Width  bit1=0  base1=MSB of Input  bit0=0  base0=LSB of Input  dbl_ovrd=off  block_type=slice
      settings: infoedit="Extracts a given range of bits from each input sample and presents it at the output.  The output type is ordinarily unsigned with binary point at zero, but can be Boolean when the slice is one bit wide.<P><P>Hardware notes: In hardware this block costs nothing."  block_version=10.1.1
  slice2 : xbsIndex_r4/Slice  nbits=1  boolean_output=on  mode=Upper Bit Location + Width  bit1=-1  base1=MSB of Input  bit0=0  base0=LSB of Input  dbl_ovrd=off  block_type=slice
      settings: infoedit="Extracts a given range of bits from each input sample and presents it at the output.  The output type is ordinarily unsigned with binary point at zero, but can be Boolean when the slice is one bit wide.<P><P>Hardware notes: In hardware this block costs nothing."  block_version=10.1.1
  dout : Outport
  of : Outport  Port=2
  wires:
  din/1 -> convert/1, slice1/1, slice2/1
  convert/1 -> dout/1
  slice1/1 -> all_1s/1, invert1/1
  invert1/1 -> all_0s/1
  slice2/1 -> all_1s/2, invert2/1
  invert2/1 -> all_0s/2
  all_0s/1 -> and/1
  all_1s/1 -> and/2
  and/1 -> of/1

== system fft_biplex_real_4x_delay_bram_test/fft_biplex_real_4x/biplex_core/fft_stage_1/butterfly_direct/convert_of1 ==
  din : Inport  OutDataType=sfix(16)  OutScaling=2^0
  all_0s : xbsIndex_r4/Logical  logical_function=NAND  inputs=2  en=off  latency=latency  precision=Full  arith_type=Unsigned  n_bits=16  bin_pt=0  align_bp=on  dbl_ovrd=off  block_type=logical
  all_1s : xbsIndex_r4/Logical  logical_function=NAND  inputs=2  en=off  latency=latency  precision=Full  arith_type=Unsigned  n_bits=16  bin_pt=0  align_bp=on  dbl_ovrd=off  block_type=logical
  and : xbsIndex_r4/Logical  logical_function=AND  inputs=2  en=off  latency=0  precision=Full  arith_type=Unsigned  n_bits=16  bin_pt=0  align_bp=on  dbl_ovrd=off  block_type=logical
  convert : xbsIndex_r4/Convert  arith_type="Signed  (2's comp)"  n_bits=bit_width_o  bin_pt=binary_point_o  quantization=Truncate  overflow=Saturate  latency=latency  dbl_ovrd=off  pipeline=on  block_type=convert
      settings: block_version=10.1.1
  invert1 : xbsIndex_r4/Inverter  en=off  latency=0  dbl_ovrd=off  block_type=inv
  invert2 : xbsIndex_r4/Inverter  en=off  latency=0  dbl_ovrd=off  block_type=inv
  slice1 : xbsIndex_r4/Slice  nbits=1  boolean_output=on  mode=Upper Bit Location + Width  bit1=0  base1=MSB of Input  bit0=0  base0=LSB of Input  dbl_ovrd=off  block_type=slice
      settings: infoedit="Extracts a given range of bits from each input sample and presents it at the output.  The output type is ordinarily unsigned with binary point at zero, but can be Boolean when the slice is one bit wide.<P><P>Hardware notes: In hardware this block costs nothing."  block_version=10.1.1
  slice2 : xbsIndex_r4/Slice  nbits=1  boolean_output=on  mode=Upper Bit Location + Width  bit1=-1  base1=MSB of Input  bit0=0  base0=LSB of Input  dbl_ovrd=off  block_type=slice
      settings: infoedit="Extracts a given range of bits from each input sample and presents it at the output.  The output type is ordinarily unsigned with binary point at zero, but can be Boolean when the slice is one bit wide.<P><P>Hardware notes: In hardware this block costs nothing."  block_version=10.1.1
  dout : Outport
  of : Outport  Port=2
  wires:
  din/1 -> convert/1, slice1/1, slice2/1
  convert/1 -> dout/1
  slice1/1 -> all_1s/1, invert1/1
  invert1/1 -> all_0s/1
  slice2/1 -> all_1s/2, invert2/1
  invert2/1 -> all_0s/2
  all_0s/1 -> and/1
  all_1s/1 -> and/2
  and/1 -> of/1

== system fft_biplex_real_4x_delay_bram_test/fft_biplex_real_4x/biplex_core/fft_stage_1/butterfly_direct/convert_of2 ==
  din : Inport  OutDataType=sfix(16)  OutScaling=2^0
  all_0s : xbsIndex_r4/Logical  logical_function=NAND  inputs=2  en=off  latency=latency  precision=Full  arith_type=Unsigned  n_bits=16  bin_pt=0  align_bp=on  dbl_ovrd=off  block_type=logical
  all_1s : xbsIndex_r4/Logical  logical_function=NAND  inputs=2  en=off  latency=latency  precision=Full  arith_type=Unsigned  n_bits=16  bin_pt=0  align_bp=on  dbl_ovrd=off  block_type=logical
  and : xbsIndex_r4/Logical  logical_function=AND  inputs=2  en=off  latency=0  precision=Full  arith_type=Unsigned  n_bits=16  bin_pt=0  align_bp=on  dbl_ovrd=off  block_type=logical
  convert : xbsIndex_r4/Convert  arith_type="Signed  (2's comp)"  n_bits=bit_width_o  bin_pt=binary_point_o  quantization=Truncate  overflow=Saturate  latency=latency  dbl_ovrd=off  pipeline=on  block_type=convert
      settings: block_version=10.1.1
  invert1 : xbsIndex_r4/Inverter  en=off  latency=0  dbl_ovrd=off  block_type=inv
  invert2 : xbsIndex_r4/Inverter  en=off  latency=0  dbl_ovrd=off  block_type=inv
  slice1 : xbsIndex_r4/Slice  nbits=1  boolean_output=on  mode=Upper Bit Location + Width  bit1=0  base1=MSB of Input  bit0=0  base0=LSB of Input  dbl_ovrd=off  block_type=slice
      settings: infoedit="Extracts a given range of bits from each input sample and presents it at the output.  The output type is ordinarily unsigned with binary point at zero, but can be Boolean when the slice is one bit wide.<P><P>Hardware notes: In hardware this block costs nothing."  block_version=10.1.1
  slice2 : xbsIndex_r4/Slice  nbits=1  boolean_output=on  mode=Upper Bit Location + Width  bit1=-1  base1=MSB of Input  bit0=0  base0=LSB of Input  dbl_ovrd=off  block_type=slice
      settings: infoedit="Extracts a given range of bits from each input sample and presents it at the output.  The output type is ordinarily unsigned with binary point at zero, but can be Boolean when the slice is one bit wide.<P><P>Hardware notes: In hardware this block costs nothing."  block_version=10.1.1
  dout : Outport
  of : Outport  Port=2
  wires:
  din/1 -> convert/1, slice1/1, slice2/1
  convert/1 -> dout/1
  slice1/1 -> all_1s/1, invert1/1
  invert1/1 -> all_0s/1
  slice2/1 -> all_1s/2, invert2/1
  invert2/1 -> all_0s/2
  all_0s/1 -> and/1
  all_1s/1 -> and/2
  and/1 -> of/1
